simulink model "Leg"  (R2025b)
settings: Solver=ode4  StartTime=0.0  StopTime=10.0  FixedStep=0.02  RelTol=1e-3
values from neighbouring files (symbols this model uses):
  g = 9.81    [SchwingenderUnterschenkel.m]
  ls = 0.4    [SchwingenderUnterschenkel.m]
  m = 4    [SchwingenderUnterschenkel.m]
  mu = 0.45    [SchwingenderUnterschenkel.m]
  omega0 = 0    [SchwingenderUnterschenkel.m]
  phi0 = interp1(timePlot.t, timePlot.phi, t0)    [SchwingenderUnterschenkel.m]
  Thetazz = 0.495    [SchwingenderUnterschenkel.m]
settings Model: Creator=cleme  LastModifiedBy=cleme

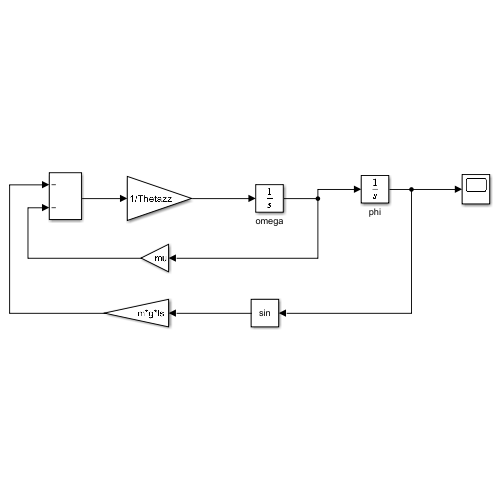
[thumbnail: Simulink's stored preview of the top-level diagram]
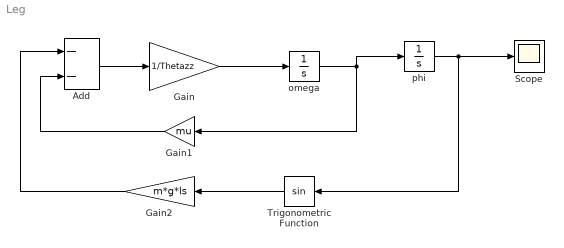
== system Leg ==
  Add : Sum  Inputs=--
  Gain : Gain  Gain=1/Thetazz
  Gain1 : Gain  Gain=mu
  Gain2 : Gain  Gain=m*g*ls
  Scope : Scope
      settings: ActiveDisplayYMinimum=-0.45841518180994417  ActiveDisplayYMaximum=0.55093502020110485
  Trigonometric Function : Trigonometry
  omega : Integrator  InitialCondition=omega0
  phi : Integrator  InitialCondition=phi0
  wires:
  Add/1 -> Gain/1
  Gain/1 -> omega/1
  omega/1 -> phi/1, Gain1/1
  Gain1/1 -> Add/2
  Gain2/1 -> Add/1
  Trigonometric Function/1 -> Gain2/1
  phi/1 -> Scope/1, Trigonometric Function/1
